simulink model "UAV3_Dynamics"  (R2026b)
settings: Solver=FixedStepDiscrete  FixedStep=0.1
settings Model: Creator=Ivan  LastModifiedBy=Ivan

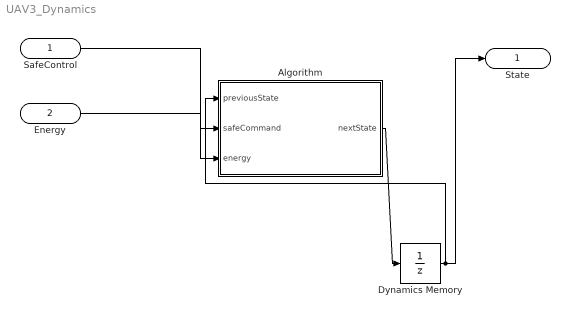
== system UAV3_Dynamics ==
  SafeControl : Inport  OutDataTypeStr=double  PortDimensions=[2 1]
  Energy : Inport  Port=2  OutDataTypeStr=double  PortDimensions=[3 1]
  Algorithm : MATLAB Function  TreatAsAtomicUnit=on
  Dynamics Memory : UnitDelay  InitialCondition=[0;0;0;0;100]  SampleTime=0.1
  State : Outport
  wires:
  Dynamics Memory/1 -> State/1, Algorithm/1(previousState)
  SafeControl/1 -> Algorithm/2(safeCommand)
  Energy/1 -> Algorithm/3(energy)
  Algorithm/1(nextState) -> Dynamics Memory/1

== matlab function UAV3_Dynamics/Algorithm ==
  data: previousState input; nextState output; safeCommand input; energy input
function nextState = dynamics_step(previousState, safeCommand, energy)
%DYNAMICS_STEP Общая двумерная модель точки массой 1 условная единица.
% State [x;y;vx;vy;battery]; discrete step = 0.1 seconds.
%#codegen
dt = 0.1;
velocity = previousState(3:4) + safeCommand*dt;
speed = sqrt(sum(velocity.^2));
if speed > 10
    velocity = velocity * (10/speed);
end
position = previousState(1:2) + velocity*dt;
battery = max(0, previousState(5)-max(0,energy(1))*dt);
nextState = [position;velocity;battery];
end
